simulink model "can2_mcu_imu_unpack"  (R2026b)
settings: Solver=VariableStepAuto
libraries: svdutilitieslib x1
settings Model: Creator=aomar  LastModifiedBy=aomar

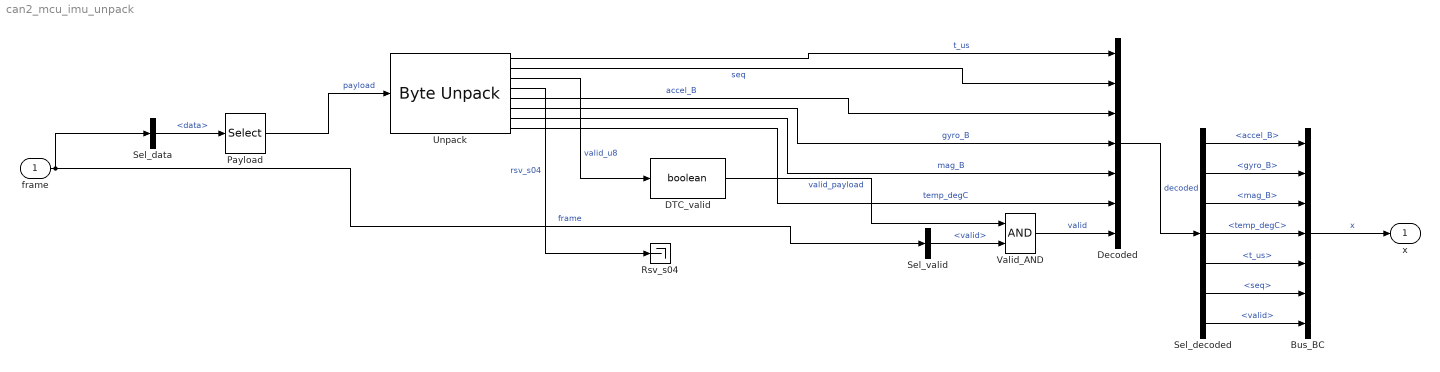
== system can2_mcu_imu_unpack ==
  frame : Inport  OutDataTypeStr=Bus: Bus_CanFrame64
  Bus_BC : BusCreator  Inputs=7  OutDataTypeStr=Bus: Bus_ImuMeas  NonVirtualBus=on
      settings: InheritFromInputs=off
  DTC_valid : DataTypeConversion  OutDataTypeStr=boolean  SaturateOnIntegerOverflow=off  RndMeth=Floor
  Decoded : BusCreator  Inputs=7
  Payload : Selector  InputPortWidth=64  IndexOptions=Index vector (dialog)  Indices=1:48  OutputSizes=1
  Rsv_s04 : Terminator
  Sel_data : BusSelector  OutputSignals=data
  Sel_decoded : BusSelector  OutputSignals=accel_B,gyro_B,mag_B,temp_degC,t_us,seq,valid
  Sel_valid : BusSelector  OutputSignals=valid
  Unpack : svdutilitieslib/Byte Unpack  dimensions={1,1,1,1,3,3,3,1}  datatypes={'uint32','uint16','uint8','uint8','single','single','single','single'}  byteAlign=1  blockPlatform=arduinoert
      settings: LibrarySourceBlock=mcblib/Signal Management/Byte Unpack
  Valid_AND : Logic  AllPortsSameDT=off  OutDataTypeStr=boolean
  x : Outport  OutDataTypeStr=Bus: Bus_ImuMeas
  wires:
  frame/1 -> Sel_valid/1, Sel_data/1  "frame"
  Sel_data/1 -> Payload/1  "<data>"
  Payload/1 -> Unpack/1  "payload"
  Unpack/1 -> Decoded/1  "t_us"
  Unpack/2 -> Decoded/2  "seq"
  Unpack/3 -> DTC_valid/1  "valid_u8"
  Unpack/4 -> Rsv_s04/1  "rsv_s04"
  Unpack/5 -> Decoded/3  "accel_B"
  Unpack/6 -> Decoded/4  "gyro_B"
  Unpack/7 -> Decoded/5  "mag_B"
  Unpack/8 -> Decoded/6  "temp_degC"
  DTC_valid/1 -> Valid_AND/1  "valid_payload"
  Sel_valid/1 -> Valid_AND/2  "<valid>"
  Valid_AND/1 -> Decoded/7  "valid"
  Decoded/1 -> Sel_decoded/1  "decoded"
  Sel_decoded/1 -> Bus_BC/1  "<accel_B>"
  Sel_decoded/2 -> Bus_BC/2  "<gyro_B>"
  Sel_decoded/3 -> Bus_BC/3  "<mag_B>"
  Sel_decoded/4 -> Bus_BC/4  "<temp_degC>"
  Sel_decoded/5 -> Bus_BC/5  "<t_us>"
  Sel_decoded/6 -> Bus_BC/6  "<seq>"
  Sel_decoded/7 -> Bus_BC/7  "<valid>"
  Bus_BC/1 -> x/1  "x"
